simulink model "snap_sys_clk_feng"  (R2019a)
settings: Solver=VariableStepDiscrete  StartTime=0.0  StopTime=10.0  RelTol=1e-3
undefined symbols (not defined in the file): datetime, posixtime
libraries: xbsIndex_r4 x5252, casper_library_misc x69, xps_library x6, casper_library_delays x3
(part 29 of 45)

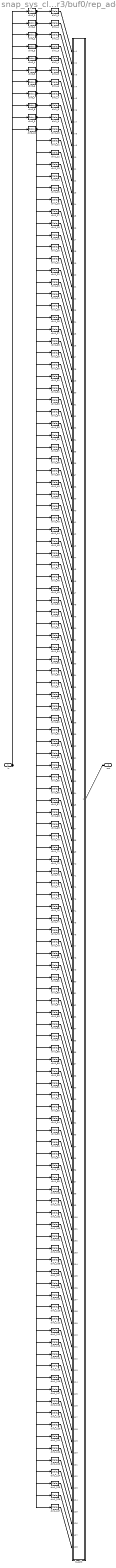
== system snap_sys_clk_feng/chan_reorder/reorder3/buf0/rep_addr ==
  in : Inport
  bussify : Subsystem  AncestorBlock=casper_library_flow_control/bus_create  mask(bus_create){inputNum=128}
      mask prompts: inputNum "Number of inputs:"
      mask init:
      | bus_create_init(gcb,...
      |     'inputNum', inputNum);
  din0_{0..10} (11 alike) : xbsIndex_r4/Delay  rst=off  infoeditControl=Selection of Reset will increase slice count due to use of real FFs and instead of SRLs  en=off  latency=1  reg_retiming=off  dbl_ovrd=off  block_type=delay
  din1_{0..127} (128 alike) : xbsIndex_r4/Delay  rst=off  infoeditControl=Selection of Reset will increase slice count due to use of real FFs and instead of SRLs  en=off  latency=1  reg_retiming=off  dbl_ovrd=off  block_type=delay
  out : Outport
  wires:
  in/1 -> din0_0/1, din0_1/1, din0_2/1, din0_3/1, din0_4/1, din0_5/1, din0_6/1, din0_7/1, din0_8/1, din0_9/1, din0_10/1
  din0_0/1 -> din1_0/1, din1_11/1, din1_22/1, din1_33/1, din1_44/1, din1_55/1, din1_66/1, din1_77/1, din1_88/1, din1_99/1, din1_110/1, din1_121/1
  din0_1/1 -> din1_1/1, din1_12/1, din1_23/1, din1_34/1, din1_45/1, din1_56/1, din1_67/1, din1_78/1, din1_89/1, din1_100/1, din1_111/1, din1_122/1
  din0_2/1 -> din1_2/1, din1_13/1, din1_24/1, din1_35/1, din1_46/1, din1_57/1, din1_68/1, din1_79/1, din1_90/1, din1_101/1, din1_112/1, din1_123/1
  din0_3/1 -> din1_3/1, din1_14/1, din1_25/1, din1_36/1, din1_47/1, din1_58/1, din1_69/1, din1_80/1, din1_91/1, din1_102/1, din1_113/1, din1_124/1
  din0_4/1 -> din1_4/1, din1_15/1, din1_26/1, din1_37/1, din1_48/1, din1_59/1, din1_70/1, din1_81/1, din1_92/1, din1_103/1, din1_114/1, din1_125/1
  din0_5/1 -> din1_5/1, din1_16/1, din1_27/1, din1_38/1, din1_49/1, din1_60/1, din1_71/1, din1_82/1, din1_93/1, din1_104/1, din1_115/1, din1_126/1
  din0_6/1 -> din1_6/1, din1_17/1, din1_28/1, din1_39/1, din1_50/1, din1_61/1, din1_72/1, din1_83/1, din1_94/1, din1_105/1, din1_116/1, din1_127/1
  din0_7/1 -> din1_7/1, din1_18/1, din1_29/1, din1_40/1, din1_51/1, din1_62/1, din1_73/1, din1_84/1, din1_95/1, din1_106/1, din1_117/1
  din0_8/1 -> din1_8/1, din1_19/1, din1_30/1, din1_41/1, din1_52/1, din1_63/1, din1_74/1, din1_85/1, din1_96/1, din1_107/1, din1_118/1
  din0_9/1 -> din1_9/1, din1_20/1, din1_31/1, din1_42/1, din1_53/1, din1_64/1, din1_75/1, din1_86/1, din1_97/1, din1_108/1, din1_119/1
  din0_10/1 -> din1_10/1, din1_21/1, din1_32/1, din1_43/1, din1_54/1, din1_65/1, din1_76/1, din1_87/1, din1_98/1, din1_109/1, din1_120/1
  din1_0/1 -> bussify/1(in1)
  din1_1/1 -> bussify/2(in2)
  din1_2/1 -> bussify/3(in3)
  din1_3/1 -> bussify/4(in4)
  din1_4/1 -> bussify/5(in5)
  din1_5/1 -> bussify/6(in6)
  din1_6/1 -> bussify/7(in7)
  din1_7/1 -> bussify/8(in8)
  din1_8/1 -> bussify/9(in9)
  din1_9/1 -> bussify/10(in10)
  din1_10/1 -> bussify/11(in11)
  din1_11/1 -> bussify/12(in12)
  din1_12/1 -> bussify/13(in13)
  din1_13/1 -> bussify/14(in14)
  din1_14/1 -> bussify/15(in15)
  din1_15/1 -> bussify/16(in16)
  din1_16/1 -> bussify/17(in17)
  din1_17/1 -> bussify/18(in18)
  din1_18/1 -> bussify/19(in19)
  din1_19/1 -> bussify/20(in20)
  din1_20/1 -> bussify/21(in21)
  din1_21/1 -> bussify/22(in22)
  din1_22/1 -> bussify/23(in23)
  din1_23/1 -> bussify/24(in24)
  din1_24/1 -> bussify/25(in25)
  din1_25/1 -> bussify/26(in26)
  din1_26/1 -> bussify/27(in27)
  din1_27/1 -> bussify/28(in28)
  din1_28/1 -> bussify/29(in29)
  din1_29/1 -> bussify/30(in30)
  din1_30/1 -> bussify/31(in31)
  din1_31/1 -> bussify/32(in32)
  din1_32/1 -> bussify/33(in33)
  din1_33/1 -> bussify/34(in34)
  din1_34/1 -> bussify/35(in35)
  din1_35/1 -> bussify/36(in36)
  din1_36/1 -> bussify/37(in37)
  din1_37/1 -> bussify/38(in38)
  din1_38/1 -> bussify/39(in39)
  din1_39/1 -> bussify/40(in40)
  din1_40/1 -> bussify/41(in41)
  din1_41/1 -> bussify/42(in42)
  din1_42/1 -> bussify/43(in43)
  din1_43/1 -> bussify/44(in44)
  din1_44/1 -> bussify/45(in45)
  din1_45/1 -> bussify/46(in46)
  din1_46/1 -> bussify/47(in47)
  din1_47/1 -> bussify/48(in48)
  din1_48/1 -> bussify/49(in49)
  din1_49/1 -> bussify/50(in50)
  din1_50/1 -> bussify/51(in51)
  din1_51/1 -> bussify/52(in52)
  din1_52/1 -> bussify/53(in53)
  din1_53/1 -> bussify/54(in54)
  din1_54/1 -> bussify/55(in55)
  din1_55/1 -> bussify/56(in56)
  din1_56/1 -> bussify/57(in57)
  din1_57/1 -> bussify/58(in58)
  din1_58/1 -> bussify/59(in59)
  din1_59/1 -> bussify/60(in60)
  din1_60/1 -> bussify/61(in61)
  din1_61/1 -> bussify/62(in62)
  din1_62/1 -> bussify/63(in63)
  din1_63/1 -> bussify/64(in64)
  din1_64/1 -> bussify/65(in65)
  din1_65/1 -> bussify/66(in66)
  din1_66/1 -> bussify/67(in67)
  din1_67/1 -> bussify/68(in68)
  din1_68/1 -> bussify/69(in69)
  din1_69/1 -> bussify/70(in70)
  din1_70/1 -> bussify/71(in71)
  din1_71/1 -> bussify/72(in72)
  din1_72/1 -> bussify/73(in73)
  din1_73/1 -> bussify/74(in74)
  din1_74/1 -> bussify/75(in75)
  din1_75/1 -> bussify/76(in76)
  din1_76/1 -> bussify/77(in77)
  din1_77/1 -> bussify/78(in78)
  din1_78/1 -> bussify/79(in79)
  din1_79/1 -> bussify/80(in80)
  din1_80/1 -> bussify/81(in81)
  din1_81/1 -> bussify/82(in82)
  din1_82/1 -> bussify/83(in83)
  din1_83/1 -> bussify/84(in84)
  din1_84/1 -> bussify/85(in85)
  din1_85/1 -> bussify/86(in86)
  din1_86/1 -> bussify/87(in87)
  din1_87/1 -> bussify/88(in88)
  din1_88/1 -> bussify/89(in89)
  din1_89/1 -> bussify/90(in90)
  din1_90/1 -> bussify/91(in91)
  din1_91/1 -> bussify/92(in92)
  din1_92/1 -> bussify/93(in93)
  din1_93/1 -> bussify/94(in94)
  din1_94/1 -> bussify/95(in95)
  din1_95/1 -> bussify/96(in96)
  din1_96/1 -> bussify/97(in97)
  din1_97/1 -> bussify/98(in98)
  din1_98/1 -> bussify/99(in99)
  din1_99/1 -> bussify/100(in100)
  din1_100/1 -> bussify/101(in101)
  din1_101/1 -> bussify/102(in102)
  din1_102/1 -> bussify/103(in103)
  din1_103/1 -> bussify/104(in104)
  din1_104/1 -> bussify/105(in105)
  din1_105/1 -> bussify/106(in106)
  din1_106/1 -> bussify/107(in107)
  din1_107/1 -> bussify/108(in108)
  din1_108/1 -> bussify/109(in109)
  din1_109/1 -> bussify/110(in110)
  din1_110/1 -> bussify/111(in111)
  din1_111/1 -> bussify/112(in112)
  din1_112/1 -> bussify/113(in113)
  din1_113/1 -> bussify/114(in114)
  din1_114/1 -> bussify/115(in115)
  din1_115/1 -> bussify/116(in116)
  din1_116/1 -> bussify/117(in117)
  din1_117/1 -> bussify/118(in118)
  din1_118/1 -> bussify/119(in119)
  din1_119/1 -> bussify/120(in120)
  din1_120/1 -> bussify/121(in121)
  din1_121/1 -> bussify/122(in122)
  din1_122/1 -> bussify/123(in123)
  din1_123/1 -> bussify/124(in124)
  din1_124/1 -> bussify/125(in125)
  din1_125/1 -> bussify/126(in126)
  din1_126/1 -> bussify/127(in127)
  din1_127/1 -> bussify/128(in128)
  bussify/1(bus_out) -> out/1

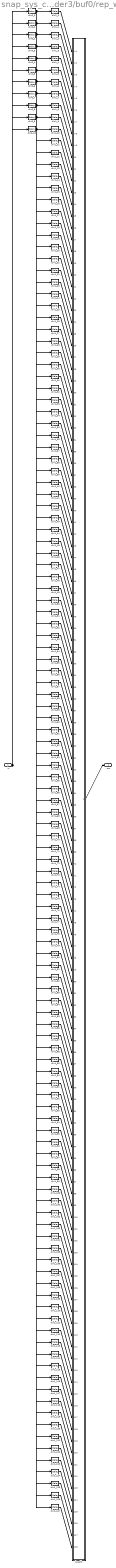
== system snap_sys_clk_feng/chan_reorder/reorder3/buf0/rep_we ==
  in : Inport
  bussify : Subsystem  AncestorBlock=casper_library_flow_control/bus_create  mask(bus_create){inputNum=128}
      mask prompts: inputNum "Number of inputs:"
      mask init:
      | bus_create_init(gcb,...
      |     'inputNum', inputNum);
  din0_{0..10} (11 alike) : xbsIndex_r4/Delay  rst=off  infoeditControl=Selection of Reset will increase slice count due to use of real FFs and instead of SRLs  en=off  latency=1  reg_retiming=off  dbl_ovrd=off  block_type=delay
  din1_{0..127} (128 alike) : xbsIndex_r4/Delay  rst=off  infoeditControl=Selection of Reset will increase slice count due to use of real FFs and instead of SRLs  en=off  latency=1  reg_retiming=off  dbl_ovrd=off  block_type=delay
  out : Outport
  wires:
  in/1 -> din0_0/1, din0_1/1, din0_2/1, din0_3/1, din0_4/1, din0_5/1, din0_6/1, din0_7/1, din0_8/1, din0_9/1, din0_10/1
  din0_0/1 -> din1_0/1, din1_11/1, din1_22/1, din1_33/1, din1_44/1, din1_55/1, din1_66/1, din1_77/1, din1_88/1, din1_99/1, din1_110/1, din1_121/1
  din0_1/1 -> din1_1/1, din1_12/1, din1_23/1, din1_34/1, din1_45/1, din1_56/1, din1_67/1, din1_78/1, din1_89/1, din1_100/1, din1_111/1, din1_122/1
  din0_2/1 -> din1_2/1, din1_13/1, din1_24/1, din1_35/1, din1_46/1, din1_57/1, din1_68/1, din1_79/1, din1_90/1, din1_101/1, din1_112/1, din1_123/1
  din0_3/1 -> din1_3/1, din1_14/1, din1_25/1, din1_36/1, din1_47/1, din1_58/1, din1_69/1, din1_80/1, din1_91/1, din1_102/1, din1_113/1, din1_124/1
  din0_4/1 -> din1_4/1, din1_15/1, din1_26/1, din1_37/1, din1_48/1, din1_59/1, din1_70/1, din1_81/1, din1_92/1, din1_103/1, din1_114/1, din1_125/1
  din0_5/1 -> din1_5/1, din1_16/1, din1_27/1, din1_38/1, din1_49/1, din1_60/1, din1_71/1, din1_82/1, din1_93/1, din1_104/1, din1_115/1, din1_126/1
  din0_6/1 -> din1_6/1, din1_17/1, din1_28/1, din1_39/1, din1_50/1, din1_61/1, din1_72/1, din1_83/1, din1_94/1, din1_105/1, din1_116/1, din1_127/1
  din0_7/1 -> din1_7/1, din1_18/1, din1_29/1, din1_40/1, din1_51/1, din1_62/1, din1_73/1, din1_84/1, din1_95/1, din1_106/1, din1_117/1
  din0_8/1 -> din1_8/1, din1_19/1, din1_30/1, din1_41/1, din1_52/1, din1_63/1, din1_74/1, din1_85/1, din1_96/1, din1_107/1, din1_118/1
  din0_9/1 -> din1_9/1, din1_20/1, din1_31/1, din1_42/1, din1_53/1, din1_64/1, din1_75/1, din1_86/1, din1_97/1, din1_108/1, din1_119/1
  din0_10/1 -> din1_10/1, din1_21/1, din1_32/1, din1_43/1, din1_54/1, din1_65/1, din1_76/1, din1_87/1, din1_98/1, din1_109/1, din1_120/1
  din1_0/1 -> bussify/1(in1)
  din1_1/1 -> bussify/2(in2)
  din1_2/1 -> bussify/3(in3)
  din1_3/1 -> bussify/4(in4)
  din1_4/1 -> bussify/5(in5)
  din1_5/1 -> bussify/6(in6)
  din1_6/1 -> bussify/7(in7)
  din1_7/1 -> bussify/8(in8)
  din1_8/1 -> bussify/9(in9)
  din1_9/1 -> bussify/10(in10)
  din1_10/1 -> bussify/11(in11)
  din1_11/1 -> bussify/12(in12)
  din1_12/1 -> bussify/13(in13)
  din1_13/1 -> bussify/14(in14)
  din1_14/1 -> bussify/15(in15)
  din1_15/1 -> bussify/16(in16)
  din1_16/1 -> bussify/17(in17)
  din1_17/1 -> bussify/18(in18)
  din1_18/1 -> bussify/19(in19)
  din1_19/1 -> bussify/20(in20)
  din1_20/1 -> bussify/21(in21)
  din1_21/1 -> bussify/22(in22)
  din1_22/1 -> bussify/23(in23)
  din1_23/1 -> bussify/24(in24)
  din1_24/1 -> bussify/25(in25)
  din1_25/1 -> bussify/26(in26)
  din1_26/1 -> bussify/27(in27)
  din1_27/1 -> bussify/28(in28)
  din1_28/1 -> bussify/29(in29)
  din1_29/1 -> bussify/30(in30)
  din1_30/1 -> bussify/31(in31)
  din1_31/1 -> bussify/32(in32)
  din1_32/1 -> bussify/33(in33)
  din1_33/1 -> bussify/34(in34)
  din1_34/1 -> bussify/35(in35)
  din1_35/1 -> bussify/36(in36)
  din1_36/1 -> bussify/37(in37)
  din1_37/1 -> bussify/38(in38)
  din1_38/1 -> bussify/39(in39)
  din1_39/1 -> bussify/40(in40)
  din1_40/1 -> bussify/41(in41)
  din1_41/1 -> bussify/42(in42)
  din1_42/1 -> bussify/43(in43)
  din1_43/1 -> bussify/44(in44)
  din1_44/1 -> bussify/45(in45)
  din1_45/1 -> bussify/46(in46)
  din1_46/1 -> bussify/47(in47)
  din1_47/1 -> bussify/48(in48)
  din1_48/1 -> bussify/49(in49)
  din1_49/1 -> bussify/50(in50)
  din1_50/1 -> bussify/51(in51)
  din1_51/1 -> bussify/52(in52)
  din1_52/1 -> bussify/53(in53)
  din1_53/1 -> bussify/54(in54)
  din1_54/1 -> bussify/55(in55)
  din1_55/1 -> bussify/56(in56)
  din1_56/1 -> bussify/57(in57)
  din1_57/1 -> bussify/58(in58)
  din1_58/1 -> bussify/59(in59)
  din1_59/1 -> bussify/60(in60)
  din1_60/1 -> bussify/61(in61)
  din1_61/1 -> bussify/62(in62)
  din1_62/1 -> bussify/63(in63)
  din1_63/1 -> bussify/64(in64)
  din1_64/1 -> bussify/65(in65)
  din1_65/1 -> bussify/66(in66)
  din1_66/1 -> bussify/67(in67)
  din1_67/1 -> bussify/68(in68)
  din1_68/1 -> bussify/69(in69)
  din1_69/1 -> bussify/70(in70)
  din1_70/1 -> bussify/71(in71)
  din1_71/1 -> bussify/72(in72)
  din1_72/1 -> bussify/73(in73)
  din1_73/1 -> bussify/74(in74)
  din1_74/1 -> bussify/75(in75)
  din1_75/1 -> bussify/76(in76)
  din1_76/1 -> bussify/77(in77)
  din1_77/1 -> bussify/78(in78)
  din1_78/1 -> bussify/79(in79)
  din1_79/1 -> bussify/80(in80)
  din1_80/1 -> bussify/81(in81)
  din1_81/1 -> bussify/82(in82)
  din1_82/1 -> bussify/83(in83)
  din1_83/1 -> bussify/84(in84)
  din1_84/1 -> bussify/85(in85)
  din1_85/1 -> bussify/86(in86)
  din1_86/1 -> bussify/87(in87)
  din1_87/1 -> bussify/88(in88)
  din1_88/1 -> bussify/89(in89)
  din1_89/1 -> bussify/90(in90)
  din1_90/1 -> bussify/91(in91)
  din1_91/1 -> bussify/92(in92)
  din1_92/1 -> bussify/93(in93)
  din1_93/1 -> bussify/94(in94)
  din1_94/1 -> bussify/95(in95)
  din1_95/1 -> bussify/96(in96)
  din1_96/1 -> bussify/97(in97)
  din1_97/1 -> bussify/98(in98)
  din1_98/1 -> bussify/99(in99)
  din1_99/1 -> bussify/100(in100)
  din1_100/1 -> bussify/101(in101)
  din1_101/1 -> bussify/102(in102)
  din1_102/1 -> bussify/103(in103)
  din1_103/1 -> bussify/104(in104)
  din1_104/1 -> bussify/105(in105)
  din1_105/1 -> bussify/106(in106)
  din1_106/1 -> bussify/107(in107)
  din1_107/1 -> bussify/108(in108)
  din1_108/1 -> bussify/109(in109)
  din1_109/1 -> bussify/110(in110)
  din1_110/1 -> bussify/111(in111)
  din1_111/1 -> bussify/112(in112)
  din1_112/1 -> bussify/113(in113)
  din1_113/1 -> bussify/114(in114)
  din1_114/1 -> bussify/115(in115)
  din1_115/1 -> bussify/116(in116)
  din1_116/1 -> bussify/117(in117)
  din1_117/1 -> bussify/118(in118)
  din1_118/1 -> bussify/119(in119)
  din1_119/1 -> bussify/120(in120)
  din1_120/1 -> bussify/121(in121)
  din1_121/1 -> bussify/122(in122)
  din1_122/1 -> bussify/123(in123)
  din1_123/1 -> bussify/124(in124)
  din1_124/1 -> bussify/125(in125)
  din1_125/1 -> bussify/126(in126)
  din1_126/1 -> bussify/127(in127)
  din1_127/1 -> bussify/128(in128)
  bussify/1(bus_out) -> out/1

== system snap_sys_clk_feng/chan_reorder/reorder3/current_map/A_bussify0 ==
  in1 : Inport
  in2 : Inport  Port=2
  in3 : Inport  Port=3
  in4 : Inport  Port=4
  in5 : Inport  Port=5
  in6 : Inport  Port=6
  in7 : Inport  Port=7
  concatenate : xbsIndex_r4/Concat  num_inputs=7  dbl_ovrd=off  block_type=concat
  reinterpret{1..7} (7 alike) : xbsIndex_r4/Reinterpret  force_arith_type=on  arith_type=Unsigned  force_bin_pt=on  bin_pt=0  block_type=reinterpret
      reinterpret1 settings: infoedit="Changes signal type without altering the binary representation.   You can changed the signal between signed and unsigned, and relocate the binary point.<br><br>Hardware notes: In hardware this block costs nothing.<br><br>Example:  Suppose the input is 6 bits wide, signed, with 2 fractional bits, and the output is forced to unsigned with 0 fractional bits.  Then an input of -2.0 (1110.00 in binary 2's complement) becomes an output of 56 (111000 in binary)."
      reinterpret2 settings: infoedit="Changes signal type without altering the binary representation.   You can changed the signal between signed and unsigned, and relocate the binary point.<br><br>Hardware notes: In hardware this block costs nothing.<br><br>Example:  Suppose the input is 6 bits wide, signed, with 2 fractional bits, and the output is forced to unsigned with 0 fractional bits.  Then an input of -2.0 (1110.00 in binary 2's complement) becomes an output of 56 (111000 in binary)."
  bus_out : Outport
  wires:
  concatenate/1 -> bus_out/1
  in1/1 -> reinterpret1/1
  reinterpret1/1 -> concatenate/1
  in2/1 -> reinterpret2/1
  reinterpret2/1 -> concatenate/2
  in3/1 -> reinterpret3/1
  reinterpret3/1 -> concatenate/3
  in4/1 -> reinterpret4/1
  reinterpret4/1 -> concatenate/4
  in5/1 -> reinterpret5/1
  reinterpret5/1 -> concatenate/5
  in6/1 -> reinterpret6/1
  reinterpret6/1 -> concatenate/6
  in7/1 -> reinterpret7/1
  reinterpret7/1 -> concatenate/7

== system snap_sys_clk_feng/chan_reorder/reorder3/current_map/B_bussify0 ==
  in1 : Inport
  in2 : Inport  Port=2
  in3 : Inport  Port=3
  in4 : Inport  Port=4
  in5 : Inport  Port=5
  in6 : Inport  Port=6
  in7 : Inport  Port=7
  concatenate : xbsIndex_r4/Concat  num_inputs=7  dbl_ovrd=off  block_type=concat
  reinterpret{1..7} (7 alike) : xbsIndex_r4/Reinterpret  force_arith_type=on  arith_type=Unsigned  force_bin_pt=on  bin_pt=0  block_type=reinterpret
      reinterpret1 settings: infoedit="Changes signal type without altering the binary representation.   You can changed the signal between signed and unsigned, and relocate the binary point.<br><br>Hardware notes: In hardware this block costs nothing.<br><br>Example:  Suppose the input is 6 bits wide, signed, with 2 fractional bits, and the output is forced to unsigned with 0 fractional bits.  Then an input of -2.0 (1110.00 in binary 2's complement) becomes an output of 56 (111000 in binary)."
      reinterpret2 settings: infoedit="Changes signal type without altering the binary representation.   You can changed the signal between signed and unsigned, and relocate the binary point.<br><br>Hardware notes: In hardware this block costs nothing.<br><br>Example:  Suppose the input is 6 bits wide, signed, with 2 fractional bits, and the output is forced to unsigned with 0 fractional bits.  Then an input of -2.0 (1110.00 in binary 2's complement) becomes an output of 56 (111000 in binary)."
  bus_out : Outport
  wires:
  concatenate/1 -> bus_out/1
  in1/1 -> reinterpret1/1
  reinterpret1/1 -> concatenate/1
  in2/1 -> reinterpret2/1
  reinterpret2/1 -> concatenate/2
  in3/1 -> reinterpret3/1
  reinterpret3/1 -> concatenate/3
  in4/1 -> reinterpret4/1
  reinterpret4/1 -> concatenate/4
  in5/1 -> reinterpret5/1
  reinterpret5/1 -> concatenate/5
  in6/1 -> reinterpret6/1
  reinterpret6/1 -> concatenate/6
  in7/1 -> reinterpret7/1
  reinterpret7/1 -> concatenate/7

== system snap_sys_clk_feng/chan_reorder/reorder3/current_map/debus_addra0 ==
  bus_in : Inport
  reinterpret{1..7} (7 alike) : xbsIndex_r4/Reinterpret  force_arith_type=on  arith_type=Unsigned  force_bin_pt=on  bin_pt=0  block_type=reinterpret
  slice1 : xbsIndex_r4/Slice  nbits=14  boolean_output=off  mode=Upper Bit Location + Width  bit1=-84  base1=MSB of Input  bit0=0  base0=LSB of Input  dbl_ovrd=off  block_type=slice
  slice2 : xbsIndex_r4/Slice  nbits=14  boolean_output=off  mode=Upper Bit Location + Width  bit1=-70  base1=MSB of Input  bit0=0  base0=LSB of Input  dbl_ovrd=off  block_type=slice
  slice3 : xbsIndex_r4/Slice  nbits=14  boolean_output=off  mode=Upper Bit Location + Width  bit1=-56  base1=MSB of Input  bit0=0  base0=LSB of Input  dbl_ovrd=off  block_type=slice
  slice4 : xbsIndex_r4/Slice  nbits=14  boolean_output=off  mode=Upper Bit Location + Width  bit1=-42  base1=MSB of Input  bit0=0  base0=LSB of Input  dbl_ovrd=off  block_type=slice
  slice5 : xbsIndex_r4/Slice  nbits=14  boolean_output=off  mode=Upper Bit Location + Width  bit1=-28  base1=MSB of Input  bit0=0  base0=LSB of Input  dbl_ovrd=off  block_type=slice
  slice6 : xbsIndex_r4/Slice  nbits=14  boolean_output=off  mode=Upper Bit Location + Width  bit1=-14  base1=MSB of Input  bit0=0  base0=LSB of Input  dbl_ovrd=off  block_type=slice
  slice7 : xbsIndex_r4/Slice  nbits=14  boolean_output=off  mode=Upper Bit Location + Width  bit1=0  base1=MSB of Input  bit0=0  base0=LSB of Input  dbl_ovrd=off  block_type=slice
  msb_out7 : Outport
  out6 : Outport  Port=2
  out5 : Outport  Port=3
  out4 : Outport  Port=4
  out3 : Outport  Port=5
  out2 : Outport  Port=6
  lsb_out1 : Outport  Port=7
  wires:
  bus_in/1 -> slice7/1, slice6/1, slice5/1, slice4/1, slice3/1, slice2/1, slice1/1
  slice7/1 -> reinterpret7/1
  reinterpret7/1 -> msb_out7/1
  slice6/1 -> reinterpret6/1
  reinterpret6/1 -> out6/1
  slice5/1 -> reinterpret5/1
  reinterpret5/1 -> out5/1
  slice4/1 -> reinterpret4/1
  reinterpret4/1 -> out4/1
  slice3/1 -> reinterpret3/1
  reinterpret3/1 -> out3/1
  slice2/1 -> reinterpret2/1
  reinterpret2/1 -> out2/1
  slice1/1 -> reinterpret1/1
  reinterpret1/1 -> lsb_out1/1

== system snap_sys_clk_feng/chan_reorder/reorder3/current_map/debus_addrb0 ==
  bus_in : Inport
  reinterpret{1..7} (7 alike) : xbsIndex_r4/Reinterpret  force_arith_type=on  arith_type=Unsigned  force_bin_pt=on  bin_pt=0  block_type=reinterpret
  slice1 : xbsIndex_r4/Slice  nbits=14  boolean_output=off  mode=Upper Bit Location + Width  bit1=-84  base1=MSB of Input  bit0=0  base0=LSB of Input  dbl_ovrd=off  block_type=slice
  slice2 : xbsIndex_r4/Slice  nbits=14  boolean_output=off  mode=Upper Bit Location + Width  bit1=-70  base1=MSB of Input  bit0=0  base0=LSB of Input  dbl_ovrd=off  block_type=slice
  slice3 : xbsIndex_r4/Slice  nbits=14  boolean_output=off  mode=Upper Bit Location + Width  bit1=-56  base1=MSB of Input  bit0=0  base0=LSB of Input  dbl_ovrd=off  block_type=slice
  slice4 : xbsIndex_r4/Slice  nbits=14  boolean_output=off  mode=Upper Bit Location + Width  bit1=-42  base1=MSB of Input  bit0=0  base0=LSB of Input  dbl_ovrd=off  block_type=slice
  slice5 : xbsIndex_r4/Slice  nbits=14  boolean_output=off  mode=Upper Bit Location + Width  bit1=-28  base1=MSB of Input  bit0=0  base0=LSB of Input  dbl_ovrd=off  block_type=slice
  slice6 : xbsIndex_r4/Slice  nbits=14  boolean_output=off  mode=Upper Bit Location + Width  bit1=-14  base1=MSB of Input  bit0=0  base0=LSB of Input  dbl_ovrd=off  block_type=slice
  slice7 : xbsIndex_r4/Slice  nbits=14  boolean_output=off  mode=Upper Bit Location + Width  bit1=0  base1=MSB of Input  bit0=0  base0=LSB of Input  dbl_ovrd=off  block_type=slice
  msb_out7 : Outport
  out6 : Outport  Port=2
  out5 : Outport  Port=3
  out4 : Outport  Port=4
  out3 : Outport  Port=5
  out2 : Outport  Port=6
  lsb_out1 : Outport  Port=7
  wires:
  bus_in/1 -> slice7/1, slice6/1, slice5/1, slice4/1, slice3/1, slice2/1, slice1/1
  slice7/1 -> reinterpret7/1
  reinterpret7/1 -> msb_out7/1
  slice6/1 -> reinterpret6/1
  reinterpret6/1 -> out6/1
  slice5/1 -> reinterpret5/1
  reinterpret5/1 -> out5/1
  slice4/1 -> reinterpret4/1
  reinterpret4/1 -> out4/1
  slice3/1 -> reinterpret3/1
  reinterpret3/1 -> out3/1
  slice2/1 -> reinterpret2/1
  reinterpret2/1 -> out2/1
  slice1/1 -> reinterpret1/1
  reinterpret1/1 -> lsb_out1/1

== system snap_sys_clk_feng/chan_reorder/reorder3/current_map/debus_dina0 ==
  bus_in : Inport
  reinterpret{1..7} (7 alike) : xbsIndex_r4/Reinterpret  force_arith_type=on  arith_type=Unsigned  force_bin_pt=on  bin_pt=0  block_type=reinterpret
  slice1 : xbsIndex_r4/Slice  nbits=2  boolean_output=off  mode=Upper Bit Location + Width  bit1=-12  base1=MSB of Input  bit0=0  base0=LSB of Input  dbl_ovrd=off  block_type=slice
  slice2 : xbsIndex_r4/Slice  nbits=2  boolean_output=off  mode=Upper Bit Location + Width  bit1=-10  base1=MSB of Input  bit0=0  base0=LSB of Input  dbl_ovrd=off  block_type=slice
  slice3 : xbsIndex_r4/Slice  nbits=2  boolean_output=off  mode=Upper Bit Location + Width  bit1=-8  base1=MSB of Input  bit0=0  base0=LSB of Input  dbl_ovrd=off  block_type=slice
  slice4 : xbsIndex_r4/Slice  nbits=2  boolean_output=off  mode=Upper Bit Location + Width  bit1=-6  base1=MSB of Input  bit0=0  base0=LSB of Input  dbl_ovrd=off  block_type=slice
  slice5 : xbsIndex_r4/Slice  nbits=2  boolean_output=off  mode=Upper Bit Location + Width  bit1=-4  base1=MSB of Input  bit0=0  base0=LSB of Input  dbl_ovrd=off  block_type=slice
  slice6 : xbsIndex_r4/Slice  nbits=2  boolean_output=off  mode=Upper Bit Location + Width  bit1=-2  base1=MSB of Input  bit0=0  base0=LSB of Input  dbl_ovrd=off  block_type=slice
  slice7 : xbsIndex_r4/Slice  nbits=2  boolean_output=off  mode=Upper Bit Location + Width  bit1=0  base1=MSB of Input  bit0=0  base0=LSB of Input  dbl_ovrd=off  block_type=slice
  msb_out7 : Outport
  out6 : Outport  Port=2
  out5 : Outport  Port=3
  out4 : Outport  Port=4
  out3 : Outport  Port=5
  out2 : Outport  Port=6
  lsb_out1 : Outport  Port=7
  wires:
  bus_in/1 -> slice7/1, slice6/1, slice5/1, slice4/1, slice3/1, slice2/1, slice1/1
  slice7/1 -> reinterpret7/1
  reinterpret7/1 -> msb_out7/1
  slice6/1 -> reinterpret6/1
  reinterpret6/1 -> out6/1
  slice5/1 -> reinterpret5/1
  reinterpret5/1 -> out5/1
  slice4/1 -> reinterpret4/1
  reinterpret4/1 -> out4/1
  slice3/1 -> reinterpret3/1
  reinterpret3/1 -> out3/1
  slice2/1 -> reinterpret2/1
  reinterpret2/1 -> out2/1
  slice1/1 -> reinterpret1/1
  reinterpret1/1 -> lsb_out1/1

== system snap_sys_clk_feng/chan_reorder/reorder3/current_map/debus_dinb0 ==
  bus_in : Inport
  reinterpret{1..7} (7 alike) : xbsIndex_r4/Reinterpret  force_arith_type=on  arith_type=Unsigned  force_bin_pt=on  bin_pt=0  block_type=reinterpret
  slice1 : xbsIndex_r4/Slice  nbits=2  boolean_output=off  mode=Upper Bit Location + Width  bit1=-12  base1=MSB of Input  bit0=0  base0=LSB of Input  dbl_ovrd=off  block_type=slice
  slice2 : xbsIndex_r4/Slice  nbits=2  boolean_output=off  mode=Upper Bit Location + Width  bit1=-10  base1=MSB of Input  bit0=0  base0=LSB of Input  dbl_ovrd=off  block_type=slice
  slice3 : xbsIndex_r4/Slice  nbits=2  boolean_output=off  mode=Upper Bit Location + Width  bit1=-8  base1=MSB of Input  bit0=0  base0=LSB of Input  dbl_ovrd=off  block_type=slice
  slice4 : xbsIndex_r4/Slice  nbits=2  boolean_output=off  mode=Upper Bit Location + Width  bit1=-6  base1=MSB of Input  bit0=0  base0=LSB of Input  dbl_ovrd=off  block_type=slice
  slice5 : xbsIndex_r4/Slice  nbits=2  boolean_output=off  mode=Upper Bit Location + Width  bit1=-4  base1=MSB of Input  bit0=0  base0=LSB of Input  dbl_ovrd=off  block_type=slice
  slice6 : xbsIndex_r4/Slice  nbits=2  boolean_output=off  mode=Upper Bit Location + Width  bit1=-2  base1=MSB of Input  bit0=0  base0=LSB of Input  dbl_ovrd=off  block_type=slice
  slice7 : xbsIndex_r4/Slice  nbits=2  boolean_output=off  mode=Upper Bit Location + Width  bit1=0  base1=MSB of Input  bit0=0  base0=LSB of Input  dbl_ovrd=off  block_type=slice
  msb_out7 : Outport
  out6 : Outport  Port=2
  out5 : Outport  Port=3
  out4 : Outport  Port=4
  out3 : Outport  Port=5
  out2 : Outport  Port=6
  lsb_out1 : Outport  Port=7
  wires:
  bus_in/1 -> slice7/1, slice6/1, slice5/1, slice4/1, slice3/1, slice2/1, slice1/1
  slice7/1 -> reinterpret7/1
  reinterpret7/1 -> msb_out7/1
  slice6/1 -> reinterpret6/1
  reinterpret6/1 -> out6/1
  slice5/1 -> reinterpret5/1
  reinterpret5/1 -> out5/1
  slice4/1 -> reinterpret4/1
  reinterpret4/1 -> out4/1
  slice3/1 -> reinterpret3/1
  reinterpret3/1 -> out3/1
  slice2/1 -> reinterpret2/1
  reinterpret2/1 -> out2/1
  slice1/1 -> reinterpret1/1
  reinterpret1/1 -> lsb_out1/1

== system snap_sys_clk_feng/chan_reorder/reorder3/current_map/debus_wea0 ==
  bus_in : Inport
  slice1 : xbsIndex_r4/Slice  nbits=1  boolean_output=on  mode=Upper Bit Location + Width  bit1=-6  base1=MSB of Input  bit0=0  base0=LSB of Input  dbl_ovrd=off  block_type=slice
  slice2 : xbsIndex_r4/Slice  nbits=1  boolean_output=on  mode=Upper Bit Location + Width  bit1=-5  base1=MSB of Input  bit0=0  base0=LSB of Input  dbl_ovrd=off  block_type=slice
  slice3 : xbsIndex_r4/Slice  nbits=1  boolean_output=on  mode=Upper Bit Location + Width  bit1=-4  base1=MSB of Input  bit0=0  base0=LSB of Input  dbl_ovrd=off  block_type=slice
  slice4 : xbsIndex_r4/Slice  nbits=1  boolean_output=on  mode=Upper Bit Location + Width  bit1=-3  base1=MSB of Input  bit0=0  base0=LSB of Input  dbl_ovrd=off  block_type=slice
  slice5 : xbsIndex_r4/Slice  nbits=1  boolean_output=on  mode=Upper Bit Location + Width  bit1=-2  base1=MSB of Input  bit0=0  base0=LSB of Input  dbl_ovrd=off  block_type=slice
  slice6 : xbsIndex_r4/Slice  nbits=1  boolean_output=on  mode=Upper Bit Location + Width  bit1=-1  base1=MSB of Input  bit0=0  base0=LSB of Input  dbl_ovrd=off  block_type=slice
  slice7 : xbsIndex_r4/Slice  nbits=1  boolean_output=on  mode=Upper Bit Location + Width  bit1=0  base1=MSB of Input  bit0=0  base0=LSB of Input  dbl_ovrd=off  block_type=slice
  msb_out7 : Outport
  out6 : Outport  Port=2
  out5 : Outport  Port=3
  out4 : Outport  Port=4
  out3 : Outport  Port=5
  out2 : Outport  Port=6
  lsb_out1 : Outport  Port=7
  wires:
  bus_in/1 -> slice7/1, slice6/1, slice5/1, slice4/1, slice3/1, slice2/1, slice1/1
  slice7/1 -> msb_out7/1
  slice6/1 -> out6/1
  slice5/1 -> out5/1
  slice4/1 -> out4/1
  slice3/1 -> out3/1
  slice2/1 -> out2/1
  slice1/1 -> lsb_out1/1

== system snap_sys_clk_feng/chan_reorder/reorder3/current_map/debus_web0 ==
  bus_in : Inport
  slice1 : xbsIndex_r4/Slice  nbits=1  boolean_output=on  mode=Upper Bit Location + Width  bit1=-6  base1=MSB of Input  bit0=0  base0=LSB of Input  dbl_ovrd=off  block_type=slice
  slice2 : xbsIndex_r4/Slice  nbits=1  boolean_output=on  mode=Upper Bit Location + Width  bit1=-5  base1=MSB of Input  bit0=0  base0=LSB of Input  dbl_ovrd=off  block_type=slice
  slice3 : xbsIndex_r4/Slice  nbits=1  boolean_output=on  mode=Upper Bit Location + Width  bit1=-4  base1=MSB of Input  bit0=0  base0=LSB of Input  dbl_ovrd=off  block_type=slice
  slice4 : xbsIndex_r4/Slice  nbits=1  boolean_output=on  mode=Upper Bit Location + Width  bit1=-3  base1=MSB of Input  bit0=0  base0=LSB of Input  dbl_ovrd=off  block_type=slice
  slice5 : xbsIndex_r4/Slice  nbits=1  boolean_output=on  mode=Upper Bit Location + Width  bit1=-2  base1=MSB of Input  bit0=0  base0=LSB of Input  dbl_ovrd=off  block_type=slice
  slice6 : xbsIndex_r4/Slice  nbits=1  boolean_output=on  mode=Upper Bit Location + Width  bit1=-1  base1=MSB of Input  bit0=0  base0=LSB of Input  dbl_ovrd=off  block_type=slice
  slice7 : xbsIndex_r4/Slice  nbits=1  boolean_output=on  mode=Upper Bit Location + Width  bit1=0  base1=MSB of Input  bit0=0  base0=LSB of Input  dbl_ovrd=off  block_type=slice
  msb_out7 : Outport
  out6 : Outport  Port=2
  out5 : Outport  Port=3
  out4 : Outport  Port=4
  out3 : Outport  Port=5
  out2 : Outport  Port=6
  lsb_out1 : Outport  Port=7
  wires:
  bus_in/1 -> slice7/1, slice6/1, slice5/1, slice4/1, slice3/1, slice2/1, slice1/1
  slice7/1 -> msb_out7/1
  slice6/1 -> out6/1
  slice5/1 -> out5/1
  slice4/1 -> out4/1
  slice3/1 -> out3/1
  slice2/1 -> out2/1
  slice1/1 -> lsb_out1/1

== system snap_sys_clk_feng/chan_reorder/reorder3/current_map/rep_addra0 ==
  in : Inport
  bussify : Subsystem  AncestorBlock=casper_library_flow_control/bus_create  mask(bus_create){inputNum=7}
      mask prompts: inputNum "Number of inputs:"
      mask init:
      | bus_create_init(gcb,...
      |     'inputNum', inputNum);
  din0_0 : xbsIndex_r4/Delay  rst=off  infoeditControl=Selection of Reset will increase slice count due to use of real FFs and instead of SRLs  en=off  latency=1  reg_retiming=on  dbl_ovrd=off  block_type=delay
  din1_0 : xbsIndex_r4/Delay  rst=off  infoeditControl=Selection of Reset will increase slice count due to use of real FFs and instead of SRLs  en=off  latency=1  reg_retiming=on  dbl_ovrd=off  block_type=delay
  din1_1 : xbsIndex_r4/Delay  rst=off  infoeditControl=Selection of Reset will increase slice count due to use of real FFs and instead of SRLs  en=off  latency=1  reg_retiming=on  dbl_ovrd=off  block_type=delay
  din2_{0..3} (4 alike) : xbsIndex_r4/Delay  rst=off  infoeditControl=Selection of Reset will increase slice count due to use of real FFs and instead of SRLs  en=off  latency=1  reg_retiming=on  dbl_ovrd=off  block_type=delay
  din3_{0..6} (7 alike) : xbsIndex_r4/Delay  rst=off  infoeditControl=Selection of Reset will increase slice count due to use of real FFs and instead of SRLs  en=off  latency=1  reg_retiming=on  dbl_ovrd=off  block_type=delay
  out : Outport
  wires:
  in/1 -> din0_0/1
  din0_0/1 -> din1_0/1, din1_1/1
  din1_0/1 -> din2_0/1, din2_2/1
  din1_1/1 -> din2_1/1, din2_3/1
  din2_0/1 -> din3_0/1, din3_4/1
  din2_1/1 -> din3_1/1, din3_5/1
  din2_2/1 -> din3_2/1, din3_6/1
  din2_3/1 -> din3_3/1
  din3_0/1 -> bussify/1(in1)
  din3_1/1 -> bussify/2(in2)
  din3_2/1 -> bussify/3(in3)
  din3_3/1 -> bussify/4(in4)
  din3_4/1 -> bussify/5(in5)
  din3_5/1 -> bussify/6(in6)
  din3_6/1 -> bussify/7(in7)
  bussify/1(bus_out) -> out/1

== system snap_sys_clk_feng/chan_reorder/reorder3/current_map/rep_addrb0 ==
  in : Inport
  bussify : Subsystem  AncestorBlock=casper_library_flow_control/bus_create  mask(bus_create){inputNum=7}
      mask prompts: inputNum "Number of inputs:"
      mask init:
      | bus_create_init(gcb,...
      |     'inputNum', inputNum);
  out : Outport
  wires:
  in/1 -> bussify/1(in1), bussify/2(in2), bussify/3(in3), bussify/4(in4), bussify/5(in5), bussify/6(in6), bussify/7(in7)
  bussify/1(bus_out) -> out/1

== system snap_sys_clk_feng/chan_reorder/reorder3/current_map/rep_wea0 ==
  in : Inport
  bussify : Subsystem  AncestorBlock=casper_library_flow_control/bus_create  mask(bus_create){inputNum=7}
      mask prompts: inputNum "Number of inputs:"
      mask init:
      | bus_create_init(gcb,...
      |     'inputNum', inputNum);
  din0_0 : xbsIndex_r4/Delay  rst=off  infoeditControl=Selection of Reset will increase slice count due to use of real FFs and instead of SRLs  en=off  latency=1  reg_retiming=off  dbl_ovrd=off  block_type=delay
  din1_0 : xbsIndex_r4/Delay  rst=off  infoeditControl=Selection of Reset will increase slice count due to use of real FFs and instead of SRLs  en=off  latency=1  reg_retiming=off  dbl_ovrd=off  block_type=delay
  din1_1 : xbsIndex_r4/Delay  rst=off  infoeditControl=Selection of Reset will increase slice count due to use of real FFs and instead of SRLs  en=off  latency=1  reg_retiming=off  dbl_ovrd=off  block_type=delay
  din2_{0..3} (4 alike) : xbsIndex_r4/Delay  rst=off  infoeditControl=Selection of Reset will increase slice count due to use of real FFs and instead of SRLs  en=off  latency=1  reg_retiming=off  dbl_ovrd=off  block_type=delay
  din3_{0..6} (7 alike) : xbsIndex_r4/Delay  rst=off  infoeditControl=Selection of Reset will increase slice count due to use of real FFs and instead of SRLs  en=off  latency=1  reg_retiming=off  dbl_ovrd=off  block_type=delay
  out : Outport
  wires:
  in/1 -> din0_0/1
  din0_0/1 -> din1_0/1, din1_1/1
  din1_0/1 -> din2_0/1, din2_2/1
  din1_1/1 -> din2_1/1, din2_3/1
  din2_0/1 -> din3_0/1, din3_4/1
  din2_1/1 -> din3_1/1, din3_5/1
  din2_2/1 -> din3_2/1, din3_6/1
  din2_3/1 -> din3_3/1
  din3_0/1 -> bussify/1(in1)
  din3_1/1 -> bussify/2(in2)
  din3_2/1 -> bussify/3(in3)
  din3_3/1 -> bussify/4(in4)
  din3_4/1 -> bussify/5(in5)
  din3_5/1 -> bussify/6(in6)
  din3_6/1 -> bussify/7(in7)
  bussify/1(bus_out) -> out/1

== system snap_sys_clk_feng/chan_reorder/reorder3/current_map/rep_web0 ==
  in : Inport
  bussify : Subsystem  AncestorBlock=casper_library_flow_control/bus_create  mask(bus_create){inputNum=7}
      mask prompts: inputNum "Number of inputs:"
      mask init:
      | bus_create_init(gcb,...
      |     'inputNum', inputNum);
  out : Outport
  wires:
  in/1 -> bussify/1(in1), bussify/2(in2), bussify/3(in3), bussify/4(in4), bussify/5(in5), bussify/6(in6), bussify/7(in7)
  bussify/1(bus_out) -> out/1

== system snap_sys_clk_feng/chan_reorder/reorder3/map/calc_add ==
  note: Use behavioural HDL
      | so that gets optimised
      | to minimum logic
  note: If reading/writing words
      | smaller than 32 bits,
      | change address so
      | that addressing is
      | big endian instead of
      | little, otherwise
      | pass through
  in : Inport
  add_sub : xbsIndex_r4/AddSub  mode=Subtraction  use_carryin=off  use_carryout=off  en=off  latency=0  precision=User Defined  arith_type=Unsigned  n_bits=max(1, log2(32/data_width))  bin_pt=0  quantization=Truncate  overflow=Wrap  use_behavioral_HDL=on  hw_selection=Fabric  pipelined=off  dbl_ovrd=off  block_type=addsub
  concat : xbsIndex_r4/Concat  num_inputs=2  dbl_ovrd=off  block_type=concat
  const : xbsIndex_r4/Constant  const=max(0, 32/data_width-1)  gui_display_data_type=Fixed-point  arith_type=Unsigned  n_bits=max(1, log2(32/data_width))  bin_pt=0  preci_type=Single  exp_width=8  frac_width=24  explicit_period=on  period=sample_rate  equ=P=C  opselect=C  inp2=PCIN>>17  opr=+  inp1=P  carry=CIN  dbl_ovrd=off  block_type=constant
      settings: block_version=11.4
  convert_addr : xbsIndex_r4/Convert  gui_display_data_type=Fixed-point  arith_type=Unsigned  n_bits=addr_width  bin_pt=0  float_type=Single  exp_bits=8  fraction_bits=24  quantization=Truncate  overflow=Wrap  en=off  latency=0  pipeline=off  dbl_ovrd=off  block_type=convert
      settings: xl_area=[0, 0, 0, 0, 0, 0, 0]
  lsw : xbsIndex_r4/Slice  nbits=max(1, log2(32/data_width))  boolean_output=off  mode=Lower Bit Location + Width  bit1=0  base1=MSB of Input  bit0=0  base0=LSB of Input  dbl_ovrd=off  block_type=slice
  manipulate : xbsIndex_r4/Constant  const=min(1, floor(32/data_width) - 1)  gui_display_data_type=Fixed-point  arith_type=Unsigned  n_bits=1  bin_pt=0  preci_type=Single  exp_width=8  frac_width=24  explicit_period=on  period=sample_rate  equ=P=C  opselect=C  inp2=PCIN>>17  opr=+  inp1=P  carry=CIN  dbl_ovrd=off  block_type=constant
      settings: block_version=11.4
  msw : xbsIndex_r4/Slice  nbits=addr_width - max(1, log2(32/data_width))  boolean_output=off  mode=Upper Bit Location + Width  bit1=0  base1=MSB of Input  bit0=0  base0=LSB of Input  dbl_ovrd=off  block_type=slice
  mux : xbsIndex_r4/Mux  inputs=2  en=off  latency=0  precision=Full  arith_type=Unsigned  n_bits=16  bin_pt=14  quantization=Truncate  overflow=Wrap  dbl_ovrd=off  block_type=mux
      settings: block_version=11.4
  out : Outport
  wires:
  convert_addr/1 -> mux/2, msw/1, lsw/1
  const/1 -> add_sub/1
  lsw/1 -> add_sub/2
  mux/1 -> out/1
  manipulate/1 -> mux/1
  concat/1 -> mux/3
  msw/1 -> concat/1
  add_sub/1 -> concat/2
  in/1 -> convert_addr/1

== system snap_sys_clk_feng/chan_reorder/reorder3/map/munge_in ==
  din : Inport
  reinterpret_out : xbsIndex_r4/Reinterpret  force_arith_type=on  arith_type=Unsigned  force_bin_pt=on  bin_pt=0  block_type=reinterpret
  dout : Outport
  wires:
  reinterpret_out/1 -> dout/1
  din/1 -> reinterpret_out/1

== system snap_sys_clk_feng/chan_reorder/reorder3/map/munge_out ==
  din : Inport
  reinterpret_out : xbsIndex_r4/Reinterpret  force_arith_type=on  arith_type=Unsigned  force_bin_pt=on  bin_pt=0  block_type=reinterpret
  dout : Outport
  wires:
  reinterpret_out/1 -> dout/1
  din/1 -> reinterpret_out/1

== system snap_sys_clk_feng/chan_reorder/reorder3/map/sim_mem ==
  addr : Inport
  data : Inport  Port=2
  we : Inport  Port=3
  Data Type Conversion : DataTypeConversion  OutDataTypeStr=single
  Data Type Conversion1 : DataTypeConversion  OutDataTypeStr=double
  Data Type Conversion2 : DataTypeConversion  OutDataTypeStr=boolean
  sfunc : M-S-Function  FunctionName=shared_bram_sim_sfunc  Parameters=depth_bits, latency, init_vals  mask{depth_bits=addr_width, latency=csp_latency, init_vals=init_vals}
      mask prompts: depth_bits "Depth (2^?):"; latency "Latency (>=1):"; init_vals "Initial values:"
      mask Callback latency:
      | latency = str2double(get_param(gcb, 'latency'));
      | if latency < 1
      |     errordlg('Cannot have latency less than one.');
      |     set_param(gcb, 'latency', '1');
      | end
  sim_addr : xbsIndex_r4/Gateway Out  inherit_from_input=off  hdl_port=off  rows=1  columns=1  UseAsDAC=off  DACChannel='1'  interface=None  automatic_assignment=on  address_offset=hex2dec('00')  intf_name=''  intf_description=''  timing_constraint=None  locs_specified=off  LOCs={}  io_standard={}  block_type=gatewayout
  sim_data : xbsIndex_r4/Gateway Out  inherit_from_input=off  hdl_port=off  rows=1  columns=1  UseAsDAC=off  DACChannel='1'  interface=None  automatic_assignment=on  address_offset=hex2dec('00')  intf_name=''  intf_description=''  timing_constraint=None  locs_specified=off  LOCs={}  io_standard={}  block_type=gatewayout
  sim_we : xbsIndex_r4/Gateway Out  inherit_from_input=off  hdl_port=off  rows=1  columns=1  UseAsDAC=off  DACChannel='1'  interface=None  automatic_assignment=on  address_offset=hex2dec('00')  intf_name=''  intf_description=''  timing_constraint=None  locs_specified=off  LOCs={}  io_standard={}  block_type=gatewayout
  data_out : Outport
  wires:
  sfunc/1 -> data_out/1  "output"
  Data Type Conversion2/1 -> sfunc/3  "we"
  Data Type Conversion1/1 -> sfunc/2  "data_in"
  Data Type Conversion/1 -> sfunc/1  "addr"
  sim_we/1 -> Data Type Conversion2/1
  sim_data/1 -> Data Type Conversion1/1
  sim_addr/1 -> Data Type Conversion/1
  we/1 -> sim_we/1
  data/1 -> sim_data/1
  addr/1 -> sim_addr/1

== system snap_sys_clk_feng/chan_reorder/reorder3/we_replicate/bussify ==
  in1 : Inport
  reinterpret1 : xbsIndex_r4/Reinterpret  force_arith_type=on  arith_type=Unsigned  force_bin_pt=on  bin_pt=0  block_type=reinterpret
      settings: infoedit="Changes signal type without altering the binary representation.   You can changed the signal between signed and unsigned, and relocate the binary point.<br><br>Hardware notes: In hardware this block costs nothing.<br><br>Example:  Suppose the input is 6 bits wide, signed, with 2 fractional bits, and the output is forced to unsigned with 0 fractional bits.  Then an input of -2.0 (1110.00 in binary 2's complement) becomes an output of 56 (111000 in binary)."
  bus_out : Outport
  wires:
  in1/1 -> reinterpret1/1
  reinterpret1/1 -> bus_out/1

== system snap_sys_clk_feng/chan_reorder/slice_duplicate/bus_convert1/bussify ==
  in1 : Inport
  in2 : Inport  Port=2
  in3 : Inport  Port=3
  in4 : Inport  Port=4
  in5 : Inport  Port=5
  in6 : Inport  Port=6
  in7 : Inport  Port=7
  in8 : Inport  Port=8
  in9 : Inport  Port=9
  in10 : Inport  Port=10
  in11 : Inport  Port=11
  in12 : Inport  Port=12
  in13 : Inport  Port=13
  in14 : Inport  Port=14
  in15 : Inport  Port=15
  in16 : Inport  Port=16
  concatenate : xbsIndex_r4/Concat  num_inputs=16  dbl_ovrd=off  block_type=concat
  reinterpret{1..16} (16 alike) : xbsIndex_r4/Reinterpret  force_arith_type=on  arith_type=Unsigned  force_bin_pt=on  bin_pt=0  block_type=reinterpret
      reinterpret1 settings: infoedit="Changes signal type without altering the binary representation.   You can changed the signal between signed and unsigned, and relocate the binary point.<br><br>Hardware notes: In hardware this block costs nothing.<br><br>Example:  Suppose the input is 6 bits wide, signed, with 2 fractional bits, and the output is forced to unsigned with 0 fractional bits.  Then an input of -2.0 (1110.00 in binary 2's complement) becomes an output of 56 (111000 in binary)."
      reinterpret2 settings: infoedit="Changes signal type without altering the binary representation.   You can changed the signal between signed and unsigned, and relocate the binary point.<br><br>Hardware notes: In hardware this block costs nothing.<br><br>Example:  Suppose the input is 6 bits wide, signed, with 2 fractional bits, and the output is forced to unsigned with 0 fractional bits.  Then an input of -2.0 (1110.00 in binary 2's complement) becomes an output of 56 (111000 in binary)."
  bus_out : Outport
  wires:
  reinterpret16/1 -> concatenate/16
  in16/1 -> reinterpret16/1
  reinterpret15/1 -> concatenate/15
  in15/1 -> reinterpret15/1
  reinterpret14/1 -> concatenate/14
  in14/1 -> reinterpret14/1
  reinterpret13/1 -> concatenate/13
  in13/1 -> reinterpret13/1
  reinterpret12/1 -> concatenate/12
  in12/1 -> reinterpret12/1
  reinterpret11/1 -> concatenate/11
  in11/1 -> reinterpret11/1
  reinterpret10/1 -> concatenate/10
  in10/1 -> reinterpret10/1
  reinterpret9/1 -> concatenate/9
  in9/1 -> reinterpret9/1
  reinterpret8/1 -> concatenate/8
  in8/1 -> reinterpret8/1
  reinterpret7/1 -> concatenate/7
  in7/1 -> reinterpret7/1
  reinterpret6/1 -> concatenate/6
  in6/1 -> reinterpret6/1
  reinterpret5/1 -> concatenate/5
  in5/1 -> reinterpret5/1
  reinterpret4/1 -> concatenate/4
  in4/1 -> reinterpret4/1
  reinterpret3/1 -> concatenate/3
  in3/1 -> reinterpret3/1
  reinterpret2/1 -> concatenate/2
  in2/1 -> reinterpret2/1
  reinterpret1/1 -> concatenate/1
  in1/1 -> reinterpret1/1
  concatenate/1 -> bus_out/1

== system snap_sys_clk_feng/chan_reorder/slice_duplicate/bus_convert1/conv1 ==
  note: (ones_bit & 1) -> round-to-even
      | (ones_bit ^ 1) -> round-to-odd
      | (sign_bit & 1)-> round-to-zero
      | (sign_bit ^ 1) -> round-to-inf
      | (X ~| 1) -> round half down
      | (X | 1) -> round half up
  in : Inport
  Concat : xbsIndex_r4/Concat  num_inputs=2  dbl_ovrd=off  block_type=concat
      settings: block_version=10.1.3
  Constant : xbsIndex_r4/Constant  const=1  gui_display_data_type=Fixed-point  arith_type=Unsigned  n_bits=1  bin_pt=0  preci_type=Single  exp_width=8  frac_width=24  explicit_period=off  period=1  equ=P=C  opselect=C  inp2=PCIN>>17  opr=+  inp1=P  carry=CIN  dbl_ovrd=off  block_type=constant
  Reinterpret : xbsIndex_r4/Reinterpret  force_arith_type=on  arith_type=Unsigned  force_bin_pt=on  bin_pt=0  block_type=reinterpret
      settings: infoedit="Changes signal type without altering the binary representation.   You can changed the signal between signed and unsigned, and relocate the binary point.<P><P>Hardware notes: In hardware this block costs nothing.<P><P>Example:  Suppose the input is 6 bits wide, signed, with 2 fractional bits, and the output is forced to unsigned with 0 fractional bits.  Then an input of -2.0 (1110.00 in binary 2's complement) becomes an output of 56 (111000 in binary)."  block_version=10.1.3
  adder : xbsIndex_r4/AddSub  mode=Addition  use_carryin=off  use_carryout=off  en=off  latency=0  precision=User Defined  arith_type="Signed  (2's comp)"  n_bits=4  bin_pt=3  quantization=Truncate  overflow=Wrap  use_behavioral_HDL=off  hw_selection=Fabric  pipelined=on  use_rpm=on  dbl_ovrd=off  block_type=addsub
      settings: xl_area=[0, 0, 0, 0, 0, 0, 0]  block_version=10.1.3
  almost_half : xbsIndex_r4/Constant  const=0  gui_display_data_type=Fixed-point  arith_type=Unsigned  n_bits=8  bin_pt=0  preci_type=Single  exp_width=8  frac_width=24  explicit_period=off  period=1  equ=P=C  opselect=C  inp2=PCIN>>17  opr=+  inp1=P  carry=CIN  dbl_ovrd=off  block_type=constant
  bit : xbsIndex_r4/Slice  nbits=1  boolean_output=off  mode=Lower Bit Location + Width  bit1=0  base1=MSB of Input  bit0=4  base0=LSB of Input  dbl_ovrd=off  block_type=slice
      settings: infoedit="Extracts a given range of bits from each input sample and presents it at the output.  The output type is ordinarily unsigned with binary point at zero, but can be Boolean when the slice is one bit wide.<P><P>Hardware notes: In hardware this block costs nothing."  block_version=10.1.3
  force1 : xbsIndex_r4/Reinterpret  force_arith_type=on  arith_type="Signed  (2's comp)"  force_bin_pt=on  bin_pt=8  block_type=reinterpret
      settings: infoedit="Changes signal type without altering the binary representation.   You can changed the signal between signed and unsigned, and relocate the binary point.<P><P>Hardware notes: In hardware this block costs nothing.<P><P>Example:  Suppose the input is 6 bits wide, signed, with 2 fractional bits, and the output is forced to unsigned with 0 fractional bits.  Then an input of -2.0 (1110.00 in binary 2's complement) becomes an output of 56 (111000 in binary)."  block_version=10.1.3
  force2 : xbsIndex_r4/Reinterpret  force_arith_type=off  arith_type="Signed  (2's comp)"  force_bin_pt=on  bin_pt=8  block_type=reinterpret
      settings: infoedit="Changes signal type without altering the binary representation.   You can changed the signal between signed and unsigned, and relocate the binary point.<P><P>Hardware notes: In hardware this block costs nothing.<P><P>Example:  Suppose the input is 6 bits wide, signed, with 2 fractional bits, and the output is forced to unsigned with 0 fractional bits.  Then an input of -2.0 (1110.00 in binary 2's complement) becomes an output of 56 (111000 in binary)."  block_version=10.1.3
  tweak_op : xbsIndex_r4/Logical  logical_function=NOR  inputs=2  en=off  latency=0  precision=Full  arith_type=Unsigned  n_bits=8  bin_pt=2  align_bp=on  dbl_ovrd=off  block_type=logical
      settings: xl_area=[0, 0, 0, 0, 0, 0, 0]
  out : Outport
  wires:
  adder/1 -> out/1
  force2/1 -> adder/2
  force1/1 -> adder/1
  Reinterpret/1 -> Concat/1
  Concat/1 -> force1/1
  in/1 -> bit/1, Reinterpret/1
  almost_half/1 -> force2/1
  bit/1 -> tweak_op/1
  Constant/1 -> tweak_op/2
  tweak_op/1 -> Concat/2
